simulink model "BattSimMode"  (R2024a)
settings: Solver=FixedStepDiscrete  StartTime=0.0  StopTime=10  FixedStep=0.01  RelTol=1e-3
model workspace (MAT data in the model file):
  ButtonDebounce_cycles = Simulink.Parameter
  ButtonDebounce_cycles.Value = 3
  ButtonDebounce_cycles.Complexity = 'real'
  ButtonDebounce_cycles.Dimensions = [1 1]
  ButtonDebounce_cycles.DataType = 'uint8'
  VersionMajor = Simulink.Parameter
  VersionMajor.Value = 0
  VersionMajor.Complexity = 'real'
  VersionMajor.Dimensions = [1 1]
  VersionMajor.DataType = 'uint8'
  VersionMinor = Simulink.Parameter
  VersionMinor.Value = 5
  VersionMinor.Complexity = 'real'
  VersionMinor.Dimensions = [1 1]
  VersionMinor.DataType = 'uint8'
  VersionPatch = Simulink.Parameter
  VersionPatch.Value = 0
  VersionPatch.Complexity = 'real'
  VersionPatch.Dimensions = [1 1]
  VersionPatch.DataType = 'uint8'
values from neighbouring files (symbols this model uses):
  ButtonDebounce_cycles = 3    [BattSimMode_data.m]
  VersionMajor = 0    [BattSimMode_data.m]
  VersionMinor = 5    [BattSimMode_data.m]
  VersionPatch = 6    [BattSimMode_data.m]
undefined symbols (not defined in the file or in its folder): QLF_ERROR, QLF_ERROR_ALIVE, QLF_ERROR_TIMEOUT, QLF_OK
Description:
  | Betriebsarten (Standby, Fernsteuerung, FAIL), Ausgang ein/aus, Tasten, Lebenszeichen und Statusbotschaft 0x121
settings Model: ParameterArgumentNames=VersionMajor,VersionMinor,VersionPatch,ButtonDebounce_cycles  Creator=danie  LastModifiedBy=danie
settings OptimizationCC: DefaultParameterBehavior=Inlined  EnhancedBackFolding=on  PassReuseOutputArgsAs=Individual arguments  ZeroExternalMemoryAtStartup=off  ZeroInternalMemoryAtStartup=off  OptimizeBlockOrder=speed  DifferentSizesBufferReuse=on  OptimizationCustomize=off  EfficientTunableParamExpr=on
settings DebuggingCC: ParameterTunabilityLossMsg=error
settings HardwareCC: ProdBitPerPointer=32  ProdBitPerSizeT=32  ProdBitPerPtrDiffT=32  ProdLargestAtomicInteger=Long  ProdLargestAtomicFloat=Double  ProdWordSize=32  ProdLongLongMode=on  ProdHWDeviceType=ARM Compatible->ARM Cortex-M
settings SFSimCC: MATLABDynamicMemAlloc=off
settings RTWCC: Description=AUTOSAR  SystemTargetFile=autosar.tlc  GenCodeOnly=on  GenerateMakefile=off  TemplateMakefile=ert_default_tmf  DataTypeReplacement=CDataTypesFixedWidth
settings CodeAppCC: ForceParamTrailComments=on  IgnoreCustomStorageClasses=off  MaxIdLength=63  OperatorAnnotations=on  SimulinkDataObjDesc=on  SFDataObjDesc=on  InsertBlockDesc=on
settings STFCustomTargetCC: MultiwordLength=256  ParMdlRefBuildCompliant=on  CompOptLevelCompliant=on  IncludeMdlTerminateFcn=off  CombineOutputUpdateFcns=on  SuppressErrorStatus=on  ERTCustomFileBanners=on  SupportNonFinite=off  SupportComplex=off  SupportContinuousTime=off  SupportNonInlinedSFcns=off  RemoveResetFunc=on  MATLABClassNameForMDSCustomization=Simulink.SoftwareTarget.ERTCustomization  AutosarCompliant=on  GRTInterface=off  LookupTableObjectStructAxisOrder=2,1,3,4,...  LUTObjectStructOrderEvenSpacing=Size,Table,Breakpoints  SystemTargetFile=autosar.tlc
settings ERTTargetCC: TargetLangStandard=C99 (ISO)  ConcurrentExecutionCompliant=off  IncludeMdlTerminateFcn=off  SuppressErrorStatus=on  SupportNonFinite=off  SupportComplex=off  ModelStepFunctionPrototypeControlCompliant=off  CPPClassGenCompliant=off  AutosarCompliant=on  LookupTableObjectStructAxisOrder=2,1,3,4,...  LUTObjectStructOrderEvenSpacing=Size,Table,Breakpoints  InlinedParameterPlacement=NonHierarchical  ERTCustomFileTemplate=example_file_process.tlc  BooleanTrueId=TRUE  BooleanFalseId=FALSE

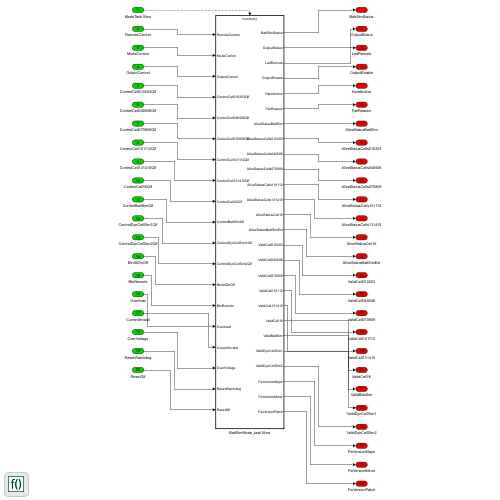
[thumbnail: Simulink's stored preview of the top-level diagram]
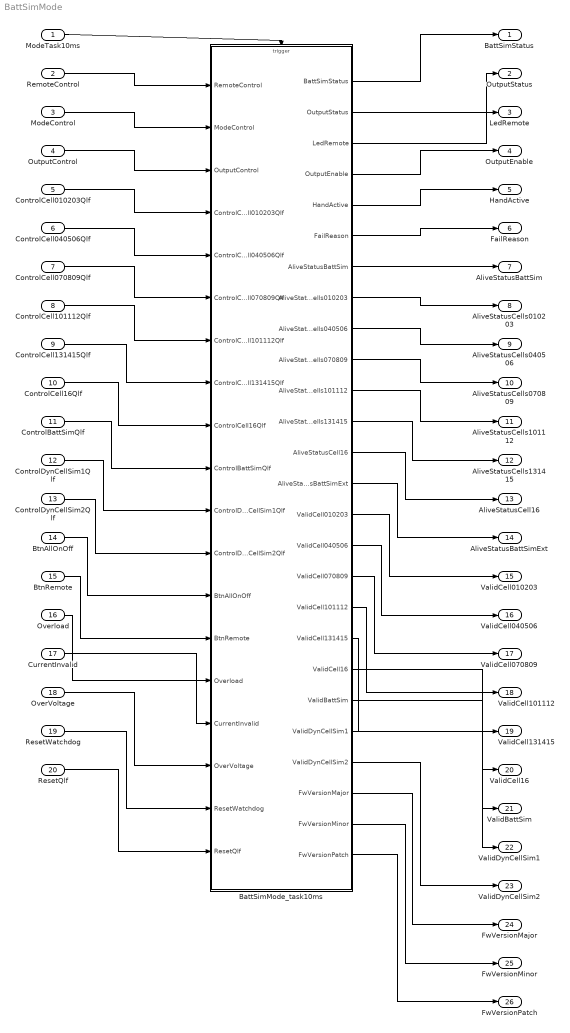
== system BattSimMode ==
  ModeTask10ms : Inport  SampleTime=0.01  OutputFunctionCall=on
  RemoteControl : Inport  Port=2  OutDataTypeStr=uint8  PortDimensions=1
  ModeControl : Inport  Port=3  OutDataTypeStr=uint8  PortDimensions=1
  OutputControl : Inport  Port=4  OutDataTypeStr=uint8  PortDimensions=1
  ControlCell010203Qlf : Inport  Port=5  OutDataTypeStr=uint8  PortDimensions=1
  ControlCell040506Qlf : Inport  Port=6  OutDataTypeStr=uint8  PortDimensions=1
  ControlCell070809Qlf : Inport  Port=7  OutDataTypeStr=uint8  PortDimensions=1
  ControlCell101112Qlf : Inport  Port=8  OutDataTypeStr=uint8  PortDimensions=1
  ControlCell131415Qlf : Inport  Port=9  OutDataTypeStr=uint8  PortDimensions=1
  ControlCell16Qlf : Inport  Port=10  OutDataTypeStr=uint8  PortDimensions=1
  ControlBattSimQlf : Inport  Port=11  OutDataTypeStr=uint8  PortDimensions=1
  ControlDynCellSim1Qlf : Inport  Port=12  OutDataTypeStr=uint8  PortDimensions=1
  ControlDynCellSim2Qlf : Inport  Port=13  OutDataTypeStr=uint8  PortDimensions=1
  BtnAllOnOff : Inport  Port=14  OutDataTypeStr=boolean  PortDimensions=1
  BtnRemote : Inport  Port=15  OutDataTypeStr=boolean  PortDimensions=1
  Overload : Inport  Port=16  OutDataTypeStr=boolean  PortDimensions=1
  CurrentInvalid : Inport  Port=17  OutDataTypeStr=boolean  PortDimensions=1
  OverVoltage : Inport  Port=18  OutDataTypeStr=boolean  PortDimensions=1
  ResetWatchdog : Inport  Port=19  OutDataTypeStr=boolean  PortDimensions=1
  ResetQlf : Inport  Port=20  OutDataTypeStr=uint8  PortDimensions=1
  BattSimMode_task10ms : Subsystem  TreatAsAtomicUnit=on
  BattSimStatus : Outport  OutDataTypeStr=uint8  PortDimensions=1
  OutputStatus : Outport  Port=2  OutDataTypeStr=uint8  PortDimensions=1
  LedRemote : Outport  Port=3  OutDataTypeStr=boolean  PortDimensions=1
  OutputEnable : Outport  Port=4  OutDataTypeStr=boolean  PortDimensions=1
  HandActive : Outport  Port=5  OutDataTypeStr=boolean  PortDimensions=1
  FailReason : Outport  Port=6  OutDataTypeStr=uint8  PortDimensions=1
  AliveStatusBattSim : Outport  Port=7  OutDataTypeStr=uint8  PortDimensions=1
  AliveStatusCells010203 : Outport  Port=8  OutDataTypeStr=uint8  PortDimensions=1
  AliveStatusCells040506 : Outport  Port=9  OutDataTypeStr=uint8  PortDimensions=1
  AliveStatusCells070809 : Outport  Port=10  OutDataTypeStr=uint8  PortDimensions=1
  AliveStatusCells101112 : Outport  Port=11  OutDataTypeStr=uint8  PortDimensions=1
  AliveStatusCells131415 : Outport  Port=12  OutDataTypeStr=uint8  PortDimensions=1
  AliveStatusCell16 : Outport  Port=13  OutDataTypeStr=uint8  PortDimensions=1
  AliveStatusBattSimExt : Outport  Port=14  OutDataTypeStr=uint8  PortDimensions=1
  ValidCell010203 : Outport  Port=15  OutDataTypeStr=boolean  PortDimensions=1
  ValidCell040506 : Outport  Port=16  OutDataTypeStr=boolean  PortDimensions=1
  ValidCell070809 : Outport  Port=17  OutDataTypeStr=boolean  PortDimensions=1
  ValidCell101112 : Outport  Port=18  OutDataTypeStr=boolean  PortDimensions=1
  ValidCell131415 : Outport  Port=19  OutDataTypeStr=boolean  PortDimensions=1
  ValidCell16 : Outport  Port=20  OutDataTypeStr=boolean  PortDimensions=1
  ValidBattSim : Outport  Port=21  OutDataTypeStr=boolean  PortDimensions=1
  ValidDynCellSim1 : Outport  Port=22  OutDataTypeStr=boolean  PortDimensions=1
  ValidDynCellSim2 : Outport  Port=23  OutDataTypeStr=boolean  PortDimensions=1
  FwVersionMajor : Outport  Port=24  OutDataTypeStr=uint8  PortDimensions=1
  FwVersionMinor : Outport  Port=25  OutDataTypeStr=uint8  PortDimensions=1
  FwVersionPatch : Outport  Port=26  OutDataTypeStr=uint8  PortDimensions=1
  wires:
  ModeTask10ms/1 -> BattSimMode_task10ms/Trigger
  RemoteControl/1 -> BattSimMode_task10ms/1(RemoteControl)
  ModeControl/1 -> BattSimMode_task10ms/2(ModeControl)
  OutputControl/1 -> BattSimMode_task10ms/3(OutputControl)
  ControlCell010203Qlf/1 -> BattSimMode_task10ms/4(ControlCell010203Qlf)
  ControlCell040506Qlf/1 -> BattSimMode_task10ms/5(ControlCell040506Qlf)
  ControlCell070809Qlf/1 -> BattSimMode_task10ms/6(ControlCell070809Qlf)
  ControlCell101112Qlf/1 -> BattSimMode_task10ms/7(ControlCell101112Qlf)
  ControlCell131415Qlf/1 -> BattSimMode_task10ms/8(ControlCell131415Qlf)
  ControlCell16Qlf/1 -> BattSimMode_task10ms/9(ControlCell16Qlf)
  ControlBattSimQlf/1 -> BattSimMode_task10ms/10(ControlBattSimQlf)
  ControlDynCellSim1Qlf/1 -> BattSimMode_task10ms/11(ControlDynCellSim1Qlf)
  ControlDynCellSim2Qlf/1 -> BattSimMode_task10ms/12(ControlDynCellSim2Qlf)
  BtnAllOnOff/1 -> BattSimMode_task10ms/13(BtnAllOnOff)
  BtnRemote/1 -> BattSimMode_task10ms/14(BtnRemote)
  Overload/1 -> BattSimMode_task10ms/15(Overload)
  CurrentInvalid/1 -> BattSimMode_task10ms/16(CurrentInvalid)
  OverVoltage/1 -> BattSimMode_task10ms/17(OverVoltage)
  ResetWatchdog/1 -> BattSimMode_task10ms/18(ResetWatchdog)
  ResetQlf/1 -> BattSimMode_task10ms/19(ResetQlf)
  BattSimMode_task10ms/1(BattSimStatus) -> BattSimStatus/1
  BattSimMode_task10ms/2(OutputStatus) -> OutputStatus/1
  BattSimMode_task10ms/3(LedRemote) -> LedRemote/1
  BattSimMode_task10ms/4(OutputEnable) -> OutputEnable/1
  BattSimMode_task10ms/5(HandActive) -> HandActive/1
  BattSimMode_task10ms/6(FailReason) -> FailReason/1
  BattSimMode_task10ms/7(AliveStatusBattSim) -> AliveStatusBattSim/1
  BattSimMode_task10ms/8(AliveStatusCells010203) -> AliveStatusCells010203/1
  BattSimMode_task10ms/9(AliveStatusCells040506) -> AliveStatusCells040506/1
  BattSimMode_task10ms/10(AliveStatusCells070809) -> AliveStatusCells070809/1
  BattSimMode_task10ms/11(AliveStatusCells101112) -> AliveStatusCells101112/1
  BattSimMode_task10ms/12(AliveStatusCells131415) -> AliveStatusCells131415/1
  BattSimMode_task10ms/13(AliveStatusCell16) -> AliveStatusCell16/1
  BattSimMode_task10ms/14(AliveStatusBattSimExt) -> AliveStatusBattSimExt/1
  BattSimMode_task10ms/15(ValidCell010203) -> ValidCell010203/1
  BattSimMode_task10ms/16(ValidCell040506) -> ValidCell040506/1
  BattSimMode_task10ms/17(ValidCell070809) -> ValidCell070809/1
  BattSimMode_task10ms/18(ValidCell101112) -> ValidCell101112/1
  BattSimMode_task10ms/19(ValidCell131415) -> ValidCell131415/1
  BattSimMode_task10ms/20(ValidCell16) -> ValidCell16/1
  BattSimMode_task10ms/21(ValidBattSim) -> ValidBattSim/1
  BattSimMode_task10ms/22(ValidDynCellSim1) -> ValidDynCellSim1/1
  BattSimMode_task10ms/23(ValidDynCellSim2) -> ValidDynCellSim2/1
  BattSimMode_task10ms/24(FwVersionMajor) -> FwVersionMajor/1
  BattSimMode_task10ms/25(FwVersionMinor) -> FwVersionMinor/1
  BattSimMode_task10ms/26(FwVersionPatch) -> FwVersionPatch/1

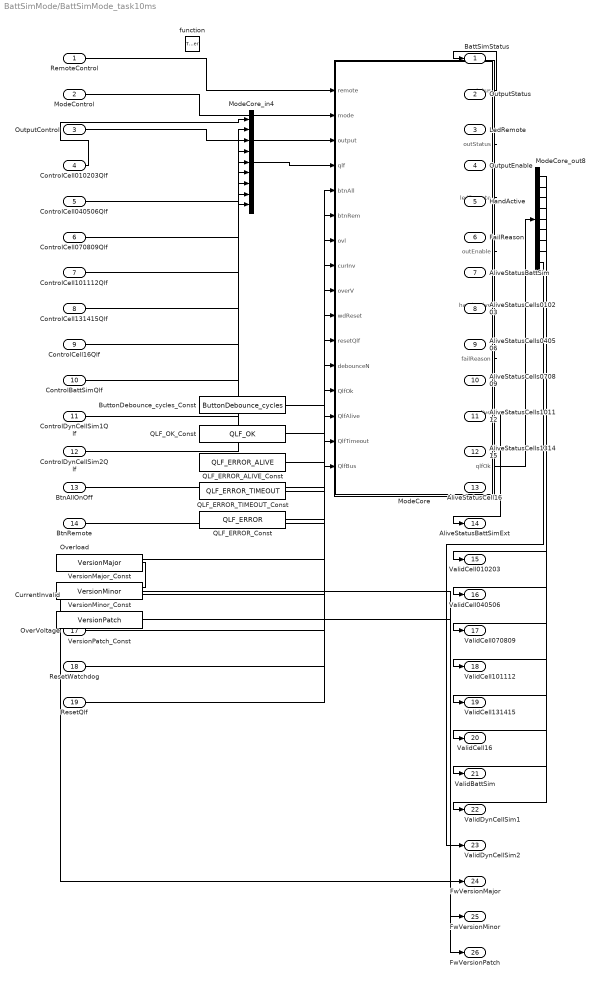
== system BattSimMode/BattSimMode_task10ms ==
  RemoteControl : Inport
  ModeControl : Inport  Port=2
  OutputControl : Inport  Port=3
  ControlCell010203Qlf : Inport  Port=4
  ControlCell040506Qlf : Inport  Port=5
  ControlCell070809Qlf : Inport  Port=6
  ControlCell101112Qlf : Inport  Port=7
  ControlCell131415Qlf : Inport  Port=8
  ControlCell16Qlf : Inport  Port=9
  ControlBattSimQlf : Inport  Port=10
  ControlDynCellSim1Qlf : Inport  Port=11
  ControlDynCellSim2Qlf : Inport  Port=12
  BtnAllOnOff : Inport  Port=13
  BtnRemote : Inport  Port=14
  Overload : Inport  Port=15
  CurrentInvalid : Inport  Port=16
  OverVoltage : Inport  Port=17
  ResetWatchdog : Inport  Port=18
  ResetQlf : Inport  Port=19
  function : TriggerPort  TriggerType=function-call  VariantControl=(inherit)  SampleTimeType=periodic  SampleTime=0.01
  ButtonDebounce_cycles_Const : Constant  Value=ButtonDebounce_cycles  OutDataTypeStr=uint8
  ModeCore : MATLAB Function  TreatAsAtomicUnit=on
  ModeCore_in4 : Mux  Inputs=9
  ModeCore_out8 : Demux  Outputs=9
  QLF_ERROR_ALIVE_Const : Constant  Value=QLF_ERROR_ALIVE  OutDataTypeStr=uint8
  QLF_ERROR_Const : Constant  Value=QLF_ERROR  OutDataTypeStr=uint8
  QLF_ERROR_TIMEOUT_Const : Constant  Value=QLF_ERROR_TIMEOUT  OutDataTypeStr=uint8
  QLF_OK_Const : Constant  Value=QLF_OK  OutDataTypeStr=uint8
  VersionMajor_Const : Constant  Value=VersionMajor  OutDataTypeStr=uint8
  VersionMinor_Const : Constant  Value=VersionMinor  OutDataTypeStr=uint8
  VersionPatch_Const : Constant  Value=VersionPatch  OutDataTypeStr=uint8
  BattSimStatus : Outport
  OutputStatus : Outport  Port=2
  LedRemote : Outport  Port=3
  OutputEnable : Outport  Port=4
  HandActive : Outport  Port=5
  FailReason : Outport  Port=6
  AliveStatusBattSim : Outport  Port=7
  AliveStatusCells010203 : Outport  Port=8
  AliveStatusCells040506 : Outport  Port=9
  AliveStatusCells070809 : Outport  Port=10
  AliveStatusCells101112 : Outport  Port=11
  AliveStatusCells131415 : Outport  Port=12
  AliveStatusCell16 : Outport  Port=13
  AliveStatusBattSimExt : Outport  Port=14
  ValidCell010203 : Outport  Port=15
  ValidCell040506 : Outport  Port=16
  ValidCell070809 : Outport  Port=17
  ValidCell101112 : Outport  Port=18
  ValidCell131415 : Outport  Port=19
  ValidCell16 : Outport  Port=20
  ValidBattSim : Outport  Port=21
  ValidDynCellSim1 : Outport  Port=22
  ValidDynCellSim2 : Outport  Port=23
  FwVersionMajor : Outport  Port=24
  FwVersionMinor : Outport  Port=25
  FwVersionPatch : Outport  Port=26
  wires:
  RemoteControl/1 -> ModeCore/1(remote)
  ModeControl/1 -> ModeCore/2(mode)
  OutputControl/1 -> ModeCore/3(output)
  ControlCell010203Qlf/1 -> ModeCore_in4/1
  ControlCell040506Qlf/1 -> ModeCore_in4/2
  ControlCell070809Qlf/1 -> ModeCore_in4/3
  ControlCell101112Qlf/1 -> ModeCore_in4/4
  ControlCell131415Qlf/1 -> ModeCore_in4/5
  ControlCell16Qlf/1 -> ModeCore_in4/6
  ControlBattSimQlf/1 -> ModeCore_in4/7
  ControlDynCellSim1Qlf/1 -> ModeCore_in4/8
  ControlDynCellSim2Qlf/1 -> ModeCore_in4/9
  ModeCore_in4/1 -> ModeCore/4(qlf)
  BtnAllOnOff/1 -> ModeCore/5(btnAll)
  BtnRemote/1 -> ModeCore/6(btnRem)
  Overload/1 -> ModeCore/7(ovl)
  CurrentInvalid/1 -> ModeCore/8(curInv)
  OverVoltage/1 -> ModeCore/9(overV)
  ResetWatchdog/1 -> ModeCore/10(wdReset)
  ResetQlf/1 -> ModeCore/11(resetQlf)
  ButtonDebounce_cycles_Const/1 -> ModeCore/12(debounceN)
  QLF_OK_Const/1 -> ModeCore/13(QlfOk)
  QLF_ERROR_ALIVE_Const/1 -> ModeCore/14(QlfAlive)
  QLF_ERROR_TIMEOUT_Const/1 -> ModeCore/15(QlfTimeout)
  QLF_ERROR_Const/1 -> ModeCore/16(QlfBus)
  ModeCore/1(status) -> BattSimStatus/1
  ModeCore/2(outStatus) -> OutputStatus/1
  ModeCore/3(ledRemote) -> LedRemote/1
  ModeCore/4(outEnable) -> OutputEnable/1
  ModeCore/5(handActive) -> HandActive/1
  ModeCore/6(failReason) -> FailReason/1
  ModeCore/7(alive) -> AliveStatusBattSim/1, AliveStatusCells010203/1, AliveStatusCells040506/1, AliveStatusCells070809/1, AliveStatusCells101112/1, AliveStatusCells131415/1, AliveStatusCell16/1, AliveStatusBattSimExt/1
  ModeCore/8(qlfOk) -> ModeCore_out8/1
  ModeCore_out8/1 -> ValidCell010203/1
  ModeCore_out8/2 -> ValidCell040506/1
  ModeCore_out8/3 -> ValidCell070809/1
  ModeCore_out8/4 -> ValidCell101112/1
  ModeCore_out8/5 -> ValidCell131415/1
  ModeCore_out8/6 -> ValidCell16/1
  ModeCore_out8/7 -> ValidBattSim/1
  ModeCore_out8/8 -> ValidDynCellSim1/1
  ModeCore_out8/9 -> ValidDynCellSim2/1
  VersionMajor_Const/1 -> FwVersionMajor/1
  VersionMinor_Const/1 -> FwVersionMinor/1
  VersionPatch_Const/1 -> FwVersionPatch/1

== matlab function BattSimMode/BattSimMode_task10ms/ModeCore ==
  data: remote input; status output; mode input; output input; qlf input; btnAll input; btnRem input; ovl input; curInv input; overV input; wdReset input; resetQlf input; debounceN input; QlfOk input; QlfAlive input; QlfTimeout input; QlfBus input; outStatus output; ledRemote output; outEnable output; handActive output; failReason output; alive output; qlfOk output
function [status, outStatus, ledRemote, outEnable, handActive, failReason, alive, qlfOk] = ModeCore(remote, mode, output, qlf, ...
    btnAll, btnRem, ovl, curInv, overV, wdReset, resetQlf, debounceN, QlfOk, QlfAlive, QlfTimeout, QlfBus)
%MODECORE Operating modes of the battery simulator, one call per 10 ms (see BattSimMode_create.m).
%#codegen
persistent st reason aliveCnt tick outBlock levA cntA levR cntR wdDone
if isempty(st)
    st = uint8(0);             % 0 STANDBY, 1 STOP, 2 RUN, 3 FAIL, 4 STANDALONE
    reason = uint8(0);
    aliveCnt = uint8(1);
    tick = uint8(0);
    outBlock = false;
    levA = false;
    cntA = uint8(0);
    levR = false;
    cntR = uint8(0);
    wdDone = false;
end

% start-up reason: the reset information is read once, as soon as its qualifier is valid
if ~wdDone && resetQlf == QlfOk
    wdDone = true;
    if wdReset && st == uint8(0) && reason == uint8(0)
        reason = uint8(4);     % this start followed a watchdog or safety reset
    end
end

[levA, cntA, pressAll] = debounce(btnAll, levA, cntA, debounceN);
[levR, cntR, pressRem] = debounce(btnRem, levR, cntR, debounceN);

% control message 0x130 (index 7 of the qualifiers): an invalid one is REMOTE=3, MODE=7, OUTPUT=3
q = qlf(7);
valid = (q == QlfOk);
r = uint8(3);
m = uint8(7);
o = uint8(3);
if valid
    r = remote;
    m = mode;
    o = output;
    if o ~= uint8(2)
        outBlock = false;
    end
end
resetCmd = (r == uint8(2)) && (m == uint8(1));
standbyCmd = (r == uint8(1)) || resetCmd;

if ovl && st ~= uint8(3)
    st = uint8(3);
    reason = uint8(3);
elseif st == uint8(2) && ~valid && (bitand(q, bitor(QlfTimeout, QlfBus)) ~= uint8(0))
    st = uint8(3);
    reason = uint8(1);
elseif st == uint8(2) && ~valid && (bitand(q, QlfAlive) ~= uint8(0))
    st = uint8(3);
    reason = uint8(2);
elseif (st == uint8(2) || st == uint8(4)) && curInv
    st = uint8(3);
    reason = uint8(5);
elseif (st == uint8(2) || st == uint8(4)) && overV
    st = uint8(3);
    reason = uint8(6);
else
    switch st
        case uint8(0)
            if pressRem || (r == uint8(2) && m == uint8(2))
                st = uint8(1);
                if reason == uint8(4)
                    reason = uint8(0);
                end
            elseif pressAll
                if curInv
                    st = uint8(3);         % hand mode is refused: the overload shut-off would be blind
                    reason = uint8(5);
                else
                    st = uint8(4);
                    if reason == uint8(4)
                        reason = uint8(0);
                    end
                end
            end
        case uint8(1)
            if pressRem || standbyCmd
                st = uint8(0);
            elseif o == uint8(2) && ~outBlock
                if curInv
                    st = uint8(3);         % RUN is refused: the overload shut-off would be blind
                    reason = uint8(5);
                else
                    st = uint8(2);
                end
            end
        case uint8(2)
            if pressRem || standbyCmd
                st = uint8(0);
            elseif pressAll
                st = uint8(1);
                outBlock = true;
            elseif o == uint8(1)
                st = uint8(1);
            end
        case uint8(4)
            if pressAll || resetCmd
                st = uint8(0);
            elseif pressRem || (r == uint8(2) && m == uint8(2))
                st = uint8(1);
                outBlock = true;           % the hand setpoints do not turn into CAN setpoints at once
            end
        otherwise
            if ~ovl && (resetCmd || pressAll)
                st = uint8(0);
                reason = uint8(0);
            end
    end
end

status = uint8(1);
if st == uint8(1) || st == uint8(2)
    status = uint8(3);
elseif st == uint8(3)
    status = uint8(5);
elseif st == uint8(4)
    status = uint8(2);
end
outStatus = uint8(1);
outEnable = (st == uint8(2)) || (st == uint8(4));
handActive = (st == uint8(4));
if outEnable
    outStatus = uint8(2);
end
ledRemote = (st == uint8(1)) || (st == uint8(2)) || ((st == uint8(3)) && (tick < uint8(20)));
failReason = reason;
alive = aliveCnt;
qlfOk = (qlf == QlfOk);

% counters for the next call: alive 1..14 once per 100 ms, tick 0..39 (200 ms blink)
if mod(tick, uint8(10)) == uint8(9)
    if aliveCnt >= uint8(14)
        aliveCnt = uint8(1);
    else
        aliveCnt = aliveCnt + uint8(1);
    end
end
if tick >= uint8(39)
    tick = uint8(0);
else
    tick = tick + uint8(1);
end

function [lvl, cnt, press] = debounce(in, lvl, cnt, n)
press = false;
if in ~= lvl
    cnt = cnt + uint8(1);
    if cnt >= n
        lvl = in;
        cnt = uint8(0);
        press = in;
    end
else
    cnt = uint8(0);
end
